simulink model "gofa_robot"  (R2023a)
settings: Solver=FixedStepAuto  StartTime=0.0  StopTime=11  FixedStep=0.001  RelTol=1e-3
undefined symbols (not defined in the file or in its folder): X, Y, Z
libraries: sm_lib x58, nesl_utility x10, slpidlib x3
(part 5 of 7)

== matlab function gofa_robot/gofa_FK_var ==
  data: x output; q1 input; y output; q2 input; q3 input; q4 input; q5 input; q6 input; z output; R output
function [x,y,z,R] = fcn(q1,q2,q3,q4,q5,q6)
d1 = 0.265;
d4 =0.47;
dee =0.101;
l3=0.444;
l4=0.110;
l6=0.08;
R=zeros(3,3);

R(1,1)= (24678615572571482867467662723121*cos(q6)*(cos(q5)*(cos(q3)*(cos(q1)*sin(q2 + pi/2) + (4967757600021511*cos(q2 + pi/2)*sin(q1))/81129638414606681695789005144064) - (4967757600021511*sin(q1))/81129638414606681695789005144064 + sin(q3)*(cos(q1)*cos(q2 + pi/2) - (4967757600021511*sin(q1)*sin(q2 + pi/2))/81129638414606681695789005144064)) + (4967757600021511*cos(q5)*(cos(q4)*sin(q1) + (4967757600021511*cos(q4)*(cos(q3)*(cos(q1)*sin(q2 + pi/2) + (4967757600021511*cos(q2 + pi/2)*sin(q1))/81129638414606681695789005144064) + sin(q3)*(cos(q1)*cos(q2 + pi/2) - (4967757600021511*sin(q1)*sin(q2 + pi/2))/81129638414606681695789005144064)))/81129638414606681695789005144064 + sin(q4)*(cos(q3)*(cos(q1)*cos(q2 + pi/2) - (4967757600021511*sin(q1)*sin(q2 + pi/2))/81129638414606681695789005144064) - sin(q3)*(cos(q1)*sin(q2 + pi/2) + (4967757600021511*cos(q2 + pi/2)*sin(q1))/81129638414606681695789005144064))))/81129638414606681695789005144064 - sin(q5)*(sin(q1)*sin(q4) - cos(q4)*(cos(q3)*(cos(q1)*cos(q2 + pi/2) - (4967757600021511*sin(q1)*sin(q2 + pi/2))/81129638414606681695789005144064) - sin(q3)*(cos(q1)*sin(q2 + pi/2) + (4967757600021511*cos(q2 + pi/2)*sin(q1))/81129638414606681695789005144064)) + (4967757600021511*sin(q4)*(cos(q3)*(cos(q1)*sin(q2 + pi/2) + (4967757600021511*cos(q2 + pi/2)*sin(q1))/81129638414606681695789005144064) + sin(q3)*(cos(q1)*cos(q2 + pi/2) - (4967757600021511*sin(q1)*sin(q2 + pi/2))/81129638414606681695789005144064)))/81129638414606681695789005144064)))/3291009114642412084309938365114701009965471731267159726697218048 - cos(q6)*(sin(q5)*(cos(q3)*(cos(q1)*sin(q2 + pi/2) + (4967757600021511*cos(q2 + pi/2)*sin(q1))/81129638414606681695789005144064) - (4967757600021511*sin(q1))/81129638414606681695789005144064 + sin(q3)*(cos(q1)*cos(q2 + pi/2) - (4967757600021511*sin(q1)*sin(q2 + pi/2))/81129638414606681695789005144064)) + (4967757600021511*sin(q5)*(cos(q4)*sin(q1) + (4967757600021511*cos(q4)*(cos(q3)*(cos(q1)*sin(q2 + pi/2) + (4967757600021511*cos(q2 + pi/2)*sin(q1))/81129638414606681695789005144064) + sin(q3)*(cos(q1)*cos(q2 + pi/2) - (4967757600021511*sin(q1)*sin(q2 + pi/2))/81129638414606681695789005144064)))/81129638414606681695789005144064 + sin(q4)*(cos(q3)*(cos(q1)*cos(q2 + pi/2) - (4967757600021511*sin(q1)*sin(q2 + pi/2))/81129638414606681695789005144064) - sin(q3)*(cos(q1)*sin(q2 + pi/2) + (4967757600021511*cos(q2 + pi/2)*sin(q1))/81129638414606681695789005144064))))/81129638414606681695789005144064 + cos(q5)*(sin(q1)*sin(q4) - cos(q4)*(cos(q3)*(cos(q1)*cos(q2 + pi/2) - (4967757600021511*sin(q1)*sin(q2 + pi/2))/81129638414606681695789005144064) - sin(q3)*(cos(q1)*sin(q2 + pi/2) + (4967757600021511*cos(q2 + pi/2)*sin(q1))/81129638414606681695789005144064)) + (4967757600021511*sin(q4)*(cos(q3)*(cos(q1)*sin(q2 + pi/2) + (4967757600021511*cos(q2 + pi/2)*sin(q1))/81129638414606681695789005144064) + sin(q3)*(cos(q1)*cos(q2 + pi/2) - (4967757600021511*sin(q1)*sin(q2 + pi/2))/81129638414606681695789005144064)))/81129638414606681695789005144064)) - (4967757600021511*sin(q6)*(cos(q5)*(cos(q3)*(cos(q1)*sin(q2 + pi/2) + (4967757600021511*cos(q2 + pi/2)*sin(q1))/81129638414606681695789005144064) - (4967757600021511*sin(q1))/81129638414606681695789005144064 + sin(q3)*(cos(q1)*cos(q2 + pi/2) - (4967757600021511*sin(q1)*sin(q2 + pi/2))/81129638414606681695789005144064)) + (4967757600021511*cos(q5)*(cos(q4)*sin(q1) + (4967757600021511*cos(q4)*(cos(q3)*(cos(q1)*sin(q2 + pi/2) + (4967757600021511*cos(q2 + pi/2)*sin(q1))/81129638414606681695789005144064) + sin(q3)*(cos(q1)*cos(q2 + pi/2) - (4967757600021511*sin(q1)*sin(q2 + pi/2))/81129638414606681695789005144064)))/81129638414606681695789005144064 + sin(q4)*(cos(q3)*(cos(q1)*cos(q2 + pi/2) - (4967757600021511*sin(q1)*sin(q2 + pi/2))/81129638414606681695789005144064) - sin(q3)*(cos(q1)*sin(q2 + pi/2) + (4967757600021511*cos(q2 + pi/2)*sin(q1))/81129638414606681695789005144064))))/81129638414606681695789005144064 - sin(q5)*(sin(q1)*sin(q4) - cos(q4)*(cos(q3)*(cos(q1)*cos(q2 + pi/2) - (4967757600021511*sin(q1)*sin(q2 + pi/2))/81129638414606681695789005144064) - sin(q3)*(cos(q1)*sin(q2 + pi/2) + (4967757600021511*cos(q2 + pi/2)*sin(q1))/81129638414606681695789005144064)) + (4967757600021511*sin(q4)*(cos(q3)*(cos(q1)*sin(q2 + pi/2) + (4967757600021511*cos(q2 + pi/2)*sin(q1))/81129638414606681695789005144064) + sin(q3)*(cos(q1)*cos(q2 + pi/2) - (4967757600021511*sin(q1)*sin(q2 + pi/2))/81129638414606681695789005144064)))/81129638414606681695789005144064)))/81129638414606681695789005144064 - (4967757600021511*sin(q6)*(sin(q5)*(cos(q3)*(cos(q1)*sin(q2 + pi/2) + (4967757600021511*cos(q2 + pi/2)*sin(q1))/81129638414606681695789005144064) - (4967757600021511*sin(q1))/81129638414606681695789005144064 + sin(q3)*(cos(q1)*cos(q2 + pi/2) - (4967757600021511*sin(q1)*sin(q2 + pi/2))/81129638414606681695789005144064)) + (4967757600021511*sin(q5)*(cos(q4)*sin(q1) + (4967757600021511*cos(q4)*(cos(q3)*(cos(q1)*sin(q2 + pi/2) + (4967757600021511*cos(q2 + pi/2)*sin(q1))/81129638414606681695789005144064) + sin(q3)*(cos(q1)*cos(q2 + pi/2) - (4967757600021511*sin(q1)*sin(q2 + pi/2))/81129638414606681695789005144064)))/81129638414606681695789005144064 + sin(q4)*(cos(q3)*(cos(q1)*cos(q2 + pi/2) - (4967757600021511*sin(q1)*sin(q2 + pi/2))/81129638414606681695789005144064) - sin(q3)*(cos(q1)*sin(q2 + pi/2) + (4967757600021511*cos(q2 + pi/2)*sin(q1))/81129638414606681695789005144064))))/81129638414606681695789005144064 + cos(q5)*(sin(q1)*sin(q4) - cos(q4)*(cos(q3)*(cos(q1)*cos(q2 + pi/2) - (4967757600021511*sin(q1)*sin(q2 + pi/2))/81129638414606681695789005144064) - sin(q3)*(cos(q1)*sin(q2 + pi/2) + (4967757600021511*cos(q2 + pi/2)*sin(q1))/81129638414606681695789005144064)) + (4967757600021511*sin(q4)*(cos(q3)*(cos(q1)*sin(q2 + pi/2) + (4967757600021511*cos(q2 + pi/2)*sin(q1))/81129638414606681695789005144064) + sin(q3)*(cos(q1)*cos(q2 + pi/2) - (4967757600021511*sin(q1)*sin(q2 + pi/2))/81129638414606681695789005144064)))/81129638414606681695789005144064)))/40564819207303340847894502572032 + (4967757600021511*cos(q6)*((24678615572571482867467662723121*sin(q1))/6582018229284824168619876730229402019930943462534319453394436096 - (4967757600021511*cos(q3)*(cos(q1)*sin(q2 + pi/2) + (4967757600021511*cos(q2 + pi/2)*sin(q1))/81129638414606681695789005144064))/81129638414606681695789005144064 + cos(q4)*sin(q1) - (4967757600021511*sin(q3)*(cos(q1)*cos(q2 + pi/2) - (4967757600021511*sin(q1)*sin(q2 + pi/2))/81129638414606681695789005144064))/81129638414606681695789005144064 + (4967757600021511*cos(q4)*(cos(q3)*(cos(q1)*sin(q2 + pi/2) + (4967757600021511*cos(q2 + pi/2)*sin(q1))/81129638414606681695789005144064) + sin(q3)*(cos(q1)*cos(q2 + pi/2) - (4967757600021511*sin(q1)*sin(q2 + pi/2))/81129638414606681695789005144064)))/81129638414606681695789005144064 + sin(q4)*(cos(q3)*(cos(q1)*cos(q2 + pi/2) - (4967757600021511*sin(q1)*sin(q2 + pi/2))/81129638414606681695789005144064) - sin(q3)*(cos(q1)*sin(q2 + pi/2) + (4967757600021511*cos(q2 + pi/2)*sin(q1))/81129638414606681695789005144064))))/40564819207303340847894502572032 - sin(q6)*((24678615572571482867467662723121*sin(q1))/6582018229284824168619876730229402019930943462534319453394436096 - (4967757600021511*cos(q3)*(cos(q1)*sin(q2 + pi/2) + (4967757600021511*cos(q2 + pi/2)*sin(q1))/81129638414606681695789005144064))/81129638414606681695789005144064 + cos(q4)*sin(q1) - (4967757600021511*sin(q3)*(cos(q1)*cos(q2 + pi/2) - (4967757600021511*sin(q1)*sin(q2 + pi/2))/81129638414606681695789005144064))/81129638414606681695789005144064 + (4967757600021511*cos(q4)*(cos(q3)*(cos(q1)*sin(q2 + pi/2) + (4967757600021511*cos(q2 + pi/2)*sin(q1))/81129638414606681695789005144064) + sin(q3)*(cos(q1)*cos(q2 + pi/2) - (4967757600021511*sin(q1)*sin(q2 + pi/2))/81129638414606681695789005144064)))/81129638414606681695789005144064 + sin(q4)*(cos(q3)*(cos(q1)*cos(q2 + pi/2) - (4967757600021511*sin(q1)*sin(q2 + pi/2))/81129638414606681695789005144064) - sin(q3)*(cos(q1)*sin(q2 + pi/2) + (4967757600021511*cos(q2 + pi/2)*sin(q1))/81129638414606681695789005144064)));
R(1,2)= sin(q6)*(sin(q5)*(cos(q3)*(cos(q1)*sin(q2 + pi/2) + (4967757600021511*cos(q2 + pi/2)*sin(q1))/81129638414606681695789005144064) - (4967757600021511*sin(q1))/81129638414606681695789005144064 + sin(q3)*(cos(q1)*cos(q2 + pi/2) - (4967757600021511*sin(q1)*sin(q2 + pi/2))/81129638414606681695789005144064)) + (4967757600021511*sin(q5)*(cos(q4)*sin(q1) + (4967757600021511*cos(q4)*(cos(q3)*(cos(q1)*sin(q2 + pi/2) + (4967757600021511*cos(q2 + pi/2)*sin(q1))/81129638414606681695789005144064) + sin(q3)*(cos(q1)*cos(q2 + pi/2) - (4967757600021511*sin(q1)*sin(q2 + pi/2))/81129638414606681695789005144064)))/81129638414606681695789005144064 + sin(q4)*(cos(q3)*(cos(q1)*cos(q2 + pi/2) - (4967757600021511*sin(q1)*sin(q2 + pi/2))/81129638414606681695789005144064) - sin(q3)*(cos(q1)*sin(q2 + pi/2) + (4967757600021511*cos(q2 + pi/2)*sin(q1))/81129638414606681695789005144064))))/81129638414606681695789005144064 + cos(q5)*(sin(q1)*sin(q4) - cos(q4)*(cos(q3)*(cos(q1)*cos(q2 + pi/2) - (4967757600021511*sin(q1)*sin(q2 + pi/2))/81129638414606681695789005144064) - sin(q3)*(cos(q1)*sin(q2 + pi/2) + (4967757600021511*cos(q2 + pi/2)*sin(q1))/81129638414606681695789005144064)) + (4967757600021511*sin(q4)*(cos(q3)*(cos(q1)*sin(q2 + pi/2) + (4967757600021511*cos(q2 + pi/2)*sin(q1))/81129638414606681695789005144064) + sin(q3)*(cos(q1)*cos(q2 + pi/2) - (4967757600021511*sin(q1)*sin(q2 + pi/2))/81129638414606681695789005144064)))/81129638414606681695789005144064)) - (4967757600021511*cos(q6)*(sin(q5)*(cos(q3)*(cos(q1)*sin(q2 + pi/2) + (4967757600021511*cos(q2 + pi/2)*sin(q1))/81129638414606681695789005144064) - (4967757600021511*sin(q1))/81129638414606681695789005144064 + sin(q3)*(cos(q1)*cos(q2 + pi/2) - (4967757600021511*sin(q1)*sin(q2 + pi/2))/81129638414606681695789005144064)) + (4967757600021511*sin(q5)*(cos(q4)*sin(q1) + (4967757600021511*cos(q4)*(cos(q3)*(cos(q1)*sin(q2 + pi/2) + (4967757600021511*cos(q2 + pi/2)*sin(q1))/81129638414606681695789005144064) + sin(q3)*(cos(q1)*cos(q2 + pi/2) - (4967757600021511*sin(q1)*sin(q2 + pi/2))/81129638414606681695789005144064)))/81129638414606681695789005144064 + sin(q4)*(cos(q3)*(cos(q1)*cos(q2 + pi/2) - (4967757600021511*sin(q1)*sin(q2 + pi/2))/81129638414606681695789005144064) - sin(q3)*(cos(q1)*sin(q2 + pi/2) + (4967757600021511*cos(q2 + pi/2)*sin(q1))/81129638414606681695789005144064))))/81129638414606681695789005144064 + cos(q5)*(sin(q1)*sin(q4) - cos(q4)*(cos(q3)*(cos(q1)*cos(q2 + pi/2) - (4967757600021511*sin(q1)*sin(q2 + pi/2))/81129638414606681695789005144064) - sin(q3)*(cos(q1)*sin(q2 + pi/2) + (4967757600021511*cos(q2 + pi/2)*sin(q1))/81129638414606681695789005144064)) + (4967757600021511*sin(q4)*(cos(q3)*(cos(q1)*sin(q2 + pi/2) + (4967757600021511*cos(q2 + pi/2)*sin(q1))/81129638414606681695789005144064) + sin(q3)*(cos(q1)*cos(q2 + pi/2) - (4967757600021511*sin(q1)*sin(q2 + pi/2))/81129638414606681695789005144064)))/81129638414606681695789005144064)))/40564819207303340847894502572032 - (24678615572571482867467662723121*sin(q6)*(cos(q5)*(cos(q3)*(cos(q1)*sin(q2 + pi/2) + (4967757600021511*cos(q2 + pi/2)*sin(q1))/81129638414606681695789005144064) - (4967757600021511*sin(q1))/81129638414606681695789005144064 + sin(q3)*(cos(q1)*cos(q2 + pi/2) - (4967757600021511*sin(q1)*sin(q2 + pi/2))/81129638414606681695789005144064)) + (4967757600021511*cos(q5)*(cos(q4)*sin(q1) + (4967757600021511*cos(q4)*(cos(q3)*(cos(q1)*sin(q2 + pi/2) + (4967757600021511*cos(q2 + pi/2)*sin(q1))/81129638414606681695789005144064) + sin(q3)*(cos(q1)*cos(q2 + pi/2) - (4967757600021511*sin(q1)*sin(q2 + pi/2))/81129638414606681695789005144064)))/81129638414606681695789005144064 + sin(q4)*(cos(q3)*(cos(q1)*cos(q2 + pi/2) - (4967757600021511*sin(q1)*sin(q2 + pi/2))/81129638414606681695789005144064) - sin(q3)*(cos(q1)*sin(q2 + pi/2) + (4967757600021511*cos(q2 + pi/2)*sin(q1))/81129638414606681695789005144064))))/81129638414606681695789005144064 - sin(q5)*(sin(q1)*sin(q4) - cos(q4)*(cos(q3)*(cos(q1)*cos(q2 + pi/2) - (4967757600021511*sin(q1)*sin(q2 + pi/2))/81129638414606681695789005144064) - sin(q3)*(cos(q1)*sin(q2 + pi/2) + (4967757600021511*cos(q2 + pi/2)*sin(q1))/81129638414606681695789005144064)) + (4967757600021511*sin(q4)*(cos(q3)*(cos(q1)*sin(q2 + pi/2) + (4967757600021511*cos(q2 + pi/2)*sin(q1))/81129638414606681695789005144064) + sin(q3)*(cos(q1)*cos(q2 + pi/2) - (4967757600021511*sin(q1)*sin(q2 + pi/2))/81129638414606681695789005144064)))/81129638414606681695789005144064)))/3291009114642412084309938365114701009965471731267159726697218048 - (4967757600021511*cos(q6)*(cos(q5)*(cos(q3)*(cos(q1)*sin(q2 + pi/2) + (4967757600021511*cos(q2 + pi/2)*sin(q1))/81129638414606681695789005144064) - (4967757600021511*sin(q1))/81129638414606681695789005144064 + sin(q3)*(cos(q1)*cos(q2 + pi/2) - (4967757600021511*sin(q1)*sin(q2 + pi/2))/81129638414606681695789005144064)) + (4967757600021511*cos(q5)*(cos(q4)*sin(q1) + (4967757600021511*cos(q4)*(cos(q3)*(cos(q1)*sin(q2 + pi/2) + (4967757600021511*cos(q2 + pi/2)*sin(q1))/81129638414606681695789005144064) + sin(q3)*(cos(q1)*cos(q2 + pi/2) - (4967757600021511*sin(q1)*sin(q2 + pi/2))/81129638414606681695789005144064)))/81129638414606681695789005144064 + sin(q4)*(cos(q3)*(cos(q1)*cos(q2 + pi/2) - (4967757600021511*sin(q1)*sin(q2 + pi/2))/81129638414606681695789005144064) - sin(q3)*(cos(q1)*sin(q2 + pi/2) + (4967757600021511*cos(q2 + pi/2)*sin(q1))/81129638414606681695789005144064))))/81129638414606681695789005144064 - sin(q5)*(sin(q1)*sin(q4) - cos(q4)*(cos(q3)*(cos(q1)*cos(q2 + pi/2) - (4967757600021511*sin(q1)*sin(q2 + pi/2))/81129638414606681695789005144064) - sin(q3)*(cos(q1)*sin(q2 + pi/2) + (4967757600021511*cos(q2 + pi/2)*sin(q1))/81129638414606681695789005144064)) + (4967757600021511*sin(q4)*(cos(q3)*(cos(q1)*sin(q2 + pi/2) + (4967757600021511*cos(q2 + pi/2)*sin(q1))/81129638414606681695789005144064) + sin(q3)*(cos(q1)*cos(q2 + pi/2) - (4967757600021511*sin(q1)*sin(q2 + pi/2))/81129638414606681695789005144064)))/81129638414606681695789005144064)))/81129638414606681695789005144064 - cos(q6)*((24678615572571482867467662723121*sin(q1))/6582018229284824168619876730229402019930943462534319453394436096 - (4967757600021511*cos(q3)*(cos(q1)*sin(q2 + pi/2) + (4967757600021511*cos(q2 + pi/2)*sin(q1))/81129638414606681695789005144064))/81129638414606681695789005144064 + cos(q4)*sin(q1) - (4967757600021511*sin(q3)*(cos(q1)*cos(q2 + pi/2) - (4967757600021511*sin(q1)*sin(q2 + pi/2))/81129638414606681695789005144064))/81129638414606681695789005144064 + (4967757600021511*cos(q4)*(cos(q3)*(cos(q1)*sin(q2 + pi/2) + (4967757600021511*cos(q2 + pi/2)*sin(q1))/81129638414606681695789005144064) + sin(q3)*(cos(q1)*cos(q2 + pi/2) - (4967757600021511*sin(q1)*sin(q2 + pi/2))/81129638414606681695789005144064)))/81129638414606681695789005144064 + sin(q4)*(cos(q3)*(cos(q1)*cos(q2 + pi/2) - (4967757600021511*sin(q1)*sin(q2 + pi/2))/81129638414606681695789005144064) - sin(q3)*(cos(q1)*sin(q2 + pi/2) + (4967757600021511*cos(q2 + pi/2)*sin(q1))/81129638414606681695789005144064))) - (4967757600021511*sin(q6)*((24678615572571482867467662723121*sin(q1))/6582018229284824168619876730229402019930943462534319453394436096 - (4967757600021511*cos(q3)*(cos(q1)*sin(q2 + pi/2) + (4967757600021511*cos(q2 + pi/2)*sin(q1))/81129638414606681695789005144064))/81129638414606681695789005144064 + cos(q4)*sin(q1) - (4967757600021511*sin(q3)*(cos(q1)*cos(q2 + pi/2) - (4967757600021511*sin(q1)*sin(q2 + pi/2))/81129638414606681695789005144064))/81129638414606681695789005144064 + (4967757600021511*cos(q4)*(cos(q3)*(cos(q1)*sin(q2 + pi/2) + (4967757600021511*cos(q2 + pi/2)*sin(q1))/81129638414606681695789005144064) + sin(q3)*(cos(q1)*cos(q2 + pi/2) - (4967757600021511*sin(q1)*sin(q2 + pi/2))/81129638414606681695789005144064)))/81129638414606681695789005144064 + sin(q4)*(cos(q3)*(cos(q1)*cos(q2 + pi/2) - (4967757600021511*sin(q1)*sin(q2 + pi/2))/81129638414606681695789005144064) - sin(q3)*(cos(q1)*sin(q2 + pi/2) + (4967757600021511*cos(q2 + pi/2)*sin(q1))/81129638414606681695789005144064))))/40564819207303340847894502572032;
R(1,3)= sin(q6)*(sin(q5)*(cos(q3)*(cos(q1)*sin(q2 + pi/2) + (4967757600021511*cos(q2 + pi/2)*sin(q1))/81129638414606681695789005144064) - (4967757600021511*sin(q1))/81129638414606681695789005144064 + sin(q3)*(cos(q1)*cos(q2 + pi/2) - (4967757600021511*sin(q1)*sin(q2 + pi/2))/81129638414606681695789005144064)) + (4967757600021511*sin(q5)*(cos(q4)*sin(q1) + (4967757600021511*cos(q4)*(cos(q3)*(cos(q1)*sin(q2 + pi/2) + (4967757600021511*cos(q2 + pi/2)*sin(q1))/81129638414606681695789005144064) + sin(q3)*(cos(q1)*cos(q2 + pi/2) - (4967757600021511*sin(q1)*sin(q2 + pi/2))/81129638414606681695789005144064)))/81129638414606681695789005144064 + sin(q4)*(cos(q3)*(cos(q1)*cos(q2 + pi/2) - (4967757600021511*sin(q1)*sin(q2 + pi/2))/81129638414606681695789005144064) - sin(q3)*(cos(q1)*sin(q2 + pi/2) + (4967757600021511*cos(q2 + pi/2)*sin(q1))/81129638414606681695789005144064))))/81129638414606681695789005144064 + cos(q5)*(sin(q1)*sin(q4) - cos(q4)*(cos(q3)*(cos(q1)*cos(q2 + pi/2) - (4967757600021511*sin(q1)*sin(q2 + pi/2))/81129638414606681695789005144064) - sin(q3)*(cos(q1)*sin(q2 + pi/2) + (4967757600021511*cos(q2 + pi/2)*sin(q1))/81129638414606681695789005144064)) + (4967757600021511*sin(q4)*(cos(q3)*(cos(q1)*sin(q2 + pi/2) + (4967757600021511*cos(q2 + pi/2)*sin(q1))/81129638414606681695789005144064) + sin(q3)*(cos(q1)*cos(q2 + pi/2) - (4967757600021511*sin(q1)*sin(q2 + pi/2))/81129638414606681695789005144064)))/81129638414606681695789005144064)) - (4967757600021511*cos(q6)*(sin(q5)*(cos(q3)*(cos(q1)*sin(q2 + pi/2) + (4967757600021511*cos(q2 + pi/2)*sin(q1))/81129638414606681695789005144064) - (4967757600021511*sin(q1))/81129638414606681695789005144064 + sin(q3)*(cos(q1)*cos(q2 + pi/2) - (4967757600021511*sin(q1)*sin(q2 + pi/2))/81129638414606681695789005144064)) + (4967757600021511*sin(q5)*(cos(q4)*sin(q1) + (4967757600021511*cos(q4)*(cos(q3)*(cos(q1)*sin(q2 + pi/2) + (4967757600021511*cos(q2 + pi/2)*sin(q1))/81129638414606681695789005144064) + sin(q3)*(cos(q1)*cos(q2 + pi/2) - (4967757600021511*sin(q1)*sin(q2 + pi/2))/81129638414606681695789005144064)))/81129638414606681695789005144064 + sin(q4)*(cos(q3)*(cos(q1)*cos(q2 + pi/2) - (4967757600021511*sin(q1)*sin(q2 + pi/2))/81129638414606681695789005144064) - sin(q3)*(cos(q1)*sin(q2 + pi/2) + (4967757600021511*cos(q2 + pi/2)*sin(q1))/81129638414606681695789005144064))))/81129638414606681695789005144064 + cos(q5)*(sin(q1)*sin(q4) - cos(q4)*(cos(q3)*(cos(q1)*cos(q2 + pi/2) - (4967757600021511*sin(q1)*sin(q2 + pi/2))/81129638414606681695789005144064) - sin(q3)*(cos(q1)*sin(q2 + pi/2) + (4967757600021511*cos(q2 + pi/2)*sin(q1))/81129638414606681695789005144064)) + (4967757600021511*sin(q4)*(cos(q3)*(cos(q1)*sin(q2 + pi/2) + (4967757600021511*cos(q2 + pi/2)*sin(q1))/81129638414606681695789005144064) + sin(q3)*(cos(q1)*cos(q2 + pi/2) - (4967757600021511*sin(q1)*sin(q2 + pi/2))/81129638414606681695789005144064)))/81129638414606681695789005144064)))/40564819207303340847894502572032 - (24678615572571482867467662723121*sin(q6)*(cos(q5)*(cos(q3)*(cos(q1)*sin(q2 + pi/2) + (4967757600021511*cos(q2 + pi/2)*sin(q1))/81129638414606681695789005144064) - (4967757600021511*sin(q1))/81129638414606681695789005144064 + sin(q3)*(cos(q1)*cos(q2 + pi/2) - (4967757600021511*sin(q1)*sin(q2 + pi/2))/81129638414606681695789005144064)) + (4967757600021511*cos(q5)*(cos(q4)*sin(q1) + (4967757600021511*cos(q4)*(cos(q3)*(cos(q1)*sin(q2 + pi/2) + (4967757600021511*cos(q2 + pi/2)*sin(q1))/81129638414606681695789005144064) + sin(q3)*(cos(q1)*cos(q2 + pi/2) - (4967757600021511*sin(q1)*sin(q2 + pi/2))/81129638414606681695789005144064)))/81129638414606681695789005144064 + sin(q4)*(cos(q3)*(cos(q1)*cos(q2 + pi/2) - (4967757600021511*sin(q1)*sin(q2 + pi/2))/81129638414606681695789005144064) - sin(q3)*(cos(q1)*sin(q2 + pi/2) + (4967757600021511*cos(q2 + pi/2)*sin(q1))/81129638414606681695789005144064))))/81129638414606681695789005144064 - sin(q5)*(sin(q1)*sin(q4) - cos(q4)*(cos(q3)*(cos(q1)*cos(q2 + pi/2) - (4967757600021511*sin(q1)*sin(q2 + pi/2))/81129638414606681695789005144064) - sin(q3)*(cos(q1)*sin(q2 + pi/2) + (4967757600021511*cos(q2 + pi/2)*sin(q1))/81129638414606681695789005144064)) + (4967757600021511*sin(q4)*(cos(q3)*(cos(q1)*sin(q2 + pi/2) + (4967757600021511*cos(q2 + pi/2)*sin(q1))/81129638414606681695789005144064) + sin(q3)*(cos(q1)*cos(q2 + pi/2) - (4967757600021511*sin(q1)*sin(q2 + pi/2))/81129638414606681695789005144064)))/81129638414606681695789005144064)))/3291009114642412084309938365114701009965471731267159726697218048 - (4967757600021511*cos(q6)*(cos(q5)*(cos(q3)*(cos(q1)*sin(q2 + pi/2) + (4967757600021511*cos(q2 + pi/2)*sin(q1))/81129638414606681695789005144064) - (4967757600021511*sin(q1))/81129638414606681695789005144064 + sin(q3)*(cos(q1)*cos(q2 + pi/2) - (4967757600021511*sin(q1)*sin(q2 + pi/2))/81129638414606681695789005144064)) + (4967757600021511*cos(q5)*(cos(q4)*sin(q1) + (4967757600021511*cos(q4)*(cos(q3)*(cos(q1)*sin(q2 + pi/2) + (4967757600021511*cos(q2 + pi/2)*sin(q1))/81129638414606681695789005144064) + sin(q3)*(cos(q1)*cos(q2 + pi/2) - (4967757600021511*sin(q1)*sin(q2 + pi/2))/81129638414606681695789005144064)))/81129638414606681695789005144064 + sin(q4)*(cos(q3)*(cos(q1)*cos(q2 + pi/2) - (4967757600021511*sin(q1)*sin(q2 + pi/2))/81129638414606681695789005144064) - sin(q3)*(cos(q1)*sin(q2 + pi/2) + (4967757600021511*cos(q2 + pi/2)*sin(q1))/81129638414606681695789005144064))))/81129638414606681695789005144064 - sin(q5)*(sin(q1)*sin(q4) - cos(q4)*(cos(q3)*(cos(q1)*cos(q2 + pi/2) - (4967757600021511*sin(q1)*sin(q2 + pi/2))/81129638414606681695789005144064) - sin(q3)*(cos(q1)*sin(q2 + pi/2) + (4967757600021511*cos(q2 + pi/2)*sin(q1))/81129638414606681695789005144064)) + (4967757600021511*sin(q4)*(cos(q3)*(cos(q1)*sin(q2 + pi/2) + (4967757600021511*cos(q2 + pi/2)*sin(q1))/81129638414606681695789005144064) + sin(q3)*(cos(q1)*cos(q2 + pi/2) - (4967757600021511*sin(q1)*sin(q2 + pi/2))/81129638414606681695789005144064)))/81129638414606681695789005144064)))/81129638414606681695789005144064 - cos(q6)*((24678615572571482867467662723121*sin(q1))/6582018229284824168619876730229402019930943462534319453394436096 - (4967757600021511*cos(q3)*(cos(q1)*sin(q2 + pi/2) + (4967757600021511*cos(q2 + pi/2)*sin(q1))/81129638414606681695789005144064))/81129638414606681695789005144064 + cos(q4)*sin(q1) - (4967757600021511*sin(q3)*(cos(q1)*cos(q2 + pi/2) - (4967757600021511*sin(q1)*sin(q2 + pi/2))/81129638414606681695789005144064))/81129638414606681695789005144064 + (4967757600021511*cos(q4)*(cos(q3)*(cos(q1)*sin(q2 + pi/2) + (4967757600021511*cos(q2 + pi/2)*sin(q1))/81129638414606681695789005144064) + sin(q3)*(cos(q1)*cos(q2 + pi/2) - (4967757600021511*sin(q1)*sin(q2 + pi/2))/81129638414606681695789005144064)))/81129638414606681695789005144064 + sin(q4)*(cos(q3)*(cos(q1)*cos(q2 + pi/2) - (4967757600021511*sin(q1)*sin(q2 + pi/2))/81129638414606681695789005144064) - sin(q3)*(cos(q1)*sin(q2 + pi/2) + (4967757600021511*cos(q2 + pi/2)*sin(q1))/81129638414606681695789005144064))) - (4967757600021511*sin(q6)*((24678615572571482867467662723121*sin(q1))/6582018229284824168619876730229402019930943462534319453394436096 - (4967757600021511*cos(q3)*(cos(q1)*sin(q2 + pi/2) + (4967757600021511*cos(q2 + pi/2)*sin(q1))/81129638414606681695789005144064))/81129638414606681695789005144064 + cos(q4)*sin(q1) - (4967757600021511*sin(q3)*(cos(q1)*cos(q2 + pi/2) - (4967757600021511*sin(q1)*sin(q2 + pi/2))/81129638414606681695789005144064))/81129638414606681695789005144064 + (4967757600021511*cos(q4)*(cos(q3)*(cos(q1)*sin(q2 + pi/2) + (4967757600021511*cos(q2 + pi/2)*sin(q1))/81129638414606681695789005144064) + sin(q3)*(cos(q1)*cos(q2 + pi/2) - (4967757600021511*sin(q1)*sin(q2 + pi/2))/81129638414606681695789005144064)))/81129638414606681695789005144064 + sin(q4)*(cos(q3)*(cos(q1)*cos(q2 + pi/2) - (4967757600021511*sin(q1)*sin(q2 + pi/2))/81129638414606681695789005144064) - sin(q3)*(cos(q1)*sin(q2 + pi/2) + (4967757600021511*cos(q2 + pi/2)*sin(q1))/81129638414606681695789005144064))))/40564819207303340847894502572032;
R(2,1)= (24678615572571482867467662723121*cos(q6)*(cos(q5)*((4967757600021511*cos(q1))/81129638414606681695789005144064 - cos(q3)*((4967757600021511*cos(q1)*cos(q2 + pi/2))/81129638414606681695789005144064 - sin(q1)*sin(q2 + pi/2)) + sin(q3)*((4967757600021511*cos(q1)*sin(q2 + pi/2))/81129638414606681695789005144064 + cos(q2 + pi/2)*sin(q1))) - (4967757600021511*cos(q5)*(cos(q1)*cos(q4) + (4967757600021511*cos(q4)*(cos(q3)*((4967757600021511*cos(q1)*cos(q2 + pi/2))/81129638414606681695789005144064 - sin(q1)*sin(q2 + pi/2)) - sin(q3)*((4967757600021511*cos(q1)*sin(q2 + pi/2))/81129638414606681695789005144064 + cos(q2 + pi/2)*sin(q1))))/81129638414606681695789005144064 - sin(q4)*(cos(q3)*((4967757600021511*cos(q1)*sin(q2 + pi/2))/81129638414606681695789005144064 + cos(q2 + pi/2)*sin(q1)) + sin(q3)*((4967757600021511*cos(q1)*cos(q2 + pi/2))/81129638414606681695789005144064 - sin(q1)*sin(q2 + pi/2)))))/81129638414606681695789005144064 + sin(q5)*(cos(q1)*sin(q4) + cos(q4)*(cos(q3)*((4967757600021511*cos(q1)*sin(q2 + pi/2))/81129638414606681695789005144064 + cos(q2 + pi/2)*sin(q1)) + sin(q3)*((4967757600021511*cos(q1)*cos(q2 + pi/2))/81129638414606681695789005144064 - sin(q1)*sin(q2 + pi/2))) + (4967757600021511*sin(q4)*(cos(q3)*((4967757600021511*cos(q1)*cos(q2 + pi/2))/81129638414606681695789005144064 - sin(q1)*sin(q2 + pi/2)) - sin(q3)*((4967757600021511*cos(q1)*sin(q2 + pi/2))/81129638414606681695789005144064 + cos(q2 + pi/2)*sin(q1))))/81129638414606681695789005144064)))/3291009114642412084309938365114701009965471731267159726697218048 - (4967757600021511*sin(q6)*(cos(q5)*((4967757600021511*cos(q1))/81129638414606681695789005144064 - cos(q3)*((4967757600021511*cos(q1)*cos(q2 + pi/2))/81129638414606681695789005144064 - sin(q1)*sin(q2 + pi/2)) + sin(q3)*((4967757600021511*cos(q1)*sin(q2 + pi/2))/81129638414606681695789005144064 + cos(q2 + pi/2)*sin(q1))) - (4967757600021511*cos(q5)*(cos(q1)*cos(q4) + (4967757600021511*cos(q4)*(cos(q3)*((4967757600021511*cos(q1)*cos(q2 + pi/2))/81129638414606681695789005144064 - sin(q1)*sin(q2 + pi/2)) - sin(q3)*((4967757600021511*cos(q1)*sin(q2 + pi/2))/81129638414606681695789005144064 + cos(q2 + pi/2)*sin(q1))))/81129638414606681695789005144064 - sin(q4)*(cos(q3)*((4967757600021511*cos(q1)*sin(q2 + pi/2))/81129638414606681695789005144064 + cos(q2 + pi/2)*sin(q1)) + sin(q3)*((4967757600021511*cos(q1)*cos(q2 + pi/2))/81129638414606681695789005144064 - sin(q1)*sin(q2 + pi/2)))))/81129638414606681695789005144064 + sin(q5)*(cos(q1)*sin(q4) + cos(q4)*(cos(q3)*((4967757600021511*cos(q1)*sin(q2 + pi/2))/81129638414606681695789005144064 + cos(q2 + pi/2)*sin(q1)) + sin(q3)*((4967757600021511*cos(q1)*cos(q2 + pi/2))/81129638414606681695789005144064 - sin(q1)*sin(q2 + pi/2))) + (4967757600021511*sin(q4)*(cos(q3)*((4967757600021511*cos(q1)*cos(q2 + pi/2))/81129638414606681695789005144064 - sin(q1)*sin(q2 + pi/2)) - sin(q3)*((4967757600021511*cos(q1)*sin(q2 + pi/2))/81129638414606681695789005144064 + cos(q2 + pi/2)*sin(q1))))/81129638414606681695789005144064)))/81129638414606681695789005144064 + cos(q6)*(cos(q5)*(cos(q1)*sin(q4) + cos(q4)*(cos(q3)*((4967757600021511*cos(q1)*sin(q2 + pi/2))/81129638414606681695789005144064 + cos(q2 + pi/2)*sin(q1)) + sin(q3)*((4967757600021511*cos(q1)*cos(q2 + pi/2))/81129638414606681695789005144064 - sin(q1)*sin(q2 + pi/2))) + (4967757600021511*sin(q4)*(cos(q3)*((4967757600021511*cos(q1)*cos(q2 + pi/2))/81129638414606681695789005144064 - sin(q1)*sin(q2 + pi/2)) - sin(q3)*((4967757600021511*cos(q1)*sin(q2 + pi/2))/81129638414606681695789005144064 + cos(q2 + pi/2)*sin(q1))))/81129638414606681695789005144064) - sin(q5)*((4967757600021511*cos(q1))/81129638414606681695789005144064 - cos(q3)*((4967757600021511*cos(q1)*cos(q2 + pi/2))/81129638414606681695789005144064 - sin(q1)*sin(q2 + pi/2)) + sin(q3)*((4967757600021511*cos(q1)*sin(q2 + pi/2))/81129638414606681695789005144064 + cos(q2 + pi/2)*sin(q1))) + (4967757600021511*sin(q5)*(cos(q1)*cos(q4) + (4967757600021511*cos(q4)*(cos(q3)*((4967757600021511*cos(q1)*cos(q2 + pi/2))/81129638414606681695789005144064 - sin(q1)*sin(q2 + pi/2)) - sin(q3)*((4967757600021511*cos(q1)*sin(q2 + pi/2))/81129638414606681695789005144064 + cos(q2 + pi/2)*sin(q1))))/81129638414606681695789005144064 - sin(q4)*(cos(q3)*((4967757600021511*cos(q1)*sin(q2 + pi/2))/81129638414606681695789005144064 + cos(q2 + pi/2)*sin(q1)) + sin(q3)*((4967757600021511*cos(q1)*cos(q2 + pi/2))/81129638414606681695789005144064 - sin(q1)*sin(q2 + pi/2)))))/81129638414606681695789005144064) + (4967757600021511*sin(q6)*(cos(q5)*(cos(q1)*sin(q4) + cos(q4)*(cos(q3)*((4967757600021511*cos(q1)*sin(q2 + pi/2))/81129638414606681695789005144064 + cos(q2 + pi/2)*sin(q1)) + sin(q3)*((4967757600021511*cos(q1)*cos(q2 + pi/2))/81129638414606681695789005144064 - sin(q1)*sin(q2 + pi/2))) + (4967757600021511*sin(q4)*(cos(q3)*((4967757600021511*cos(q1)*cos(q2 + pi/2))/81129638414606681695789005144064 - sin(q1)*sin(q2 + pi/2)) - sin(q3)*((4967757600021511*cos(q1)*sin(q2 + pi/2))/81129638414606681695789005144064 + cos(q2 + pi/2)*sin(q1))))/81129638414606681695789005144064) - sin(q5)*((4967757600021511*cos(q1))/81129638414606681695789005144064 - cos(q3)*((4967757600021511*cos(q1)*cos(q2 + pi/2))/81129638414606681695789005144064 - sin(q1)*sin(q2 + pi/2)) + sin(q3)*((4967757600021511*cos(q1)*sin(q2 + pi/2))/81129638414606681695789005144064 + cos(q2 + pi/2)*sin(q1))) + (4967757600021511*sin(q5)*(cos(q1)*cos(q4) + (4967757600021511*cos(q4)*(cos(q3)*((4967757600021511*cos(q1)*cos(q2 + pi/2))/81129638414606681695789005144064 - sin(q1)*sin(q2 + pi/2)) - sin(q3)*((4967757600021511*cos(q1)*sin(q2 + pi/2))/81129638414606681695789005144064 + cos(q2 + pi/2)*sin(q1))))/81129638414606681695789005144064 - sin(q4)*(cos(q3)*((4967757600021511*cos(q1)*sin(q2 + pi/2))/81129638414606681695789005144064 + cos(q2 + pi/2)*sin(q1)) + sin(q3)*((4967757600021511*cos(q1)*cos(q2 + pi/2))/81129638414606681695789005144064 - sin(q1)*sin(q2 + pi/2)))))/81129638414606681695789005144064))/40564819207303340847894502572032 - (4967757600021511*cos(q6)*((24678615572571482867467662723121*cos(q1))/6582018229284824168619876730229402019930943462534319453394436096 + cos(q1)*cos(q4) - (4967757600021511*cos(q3)*((4967757600021511*cos(q1)*cos(q2 + pi/2))/81129638414606681695789005144064 - sin(q1)*sin(q2 + pi/2)))/81129638414606681695789005144064 + (4967757600021511*sin(q3)*((4967757600021511*cos(q1)*sin(q2 + pi/2))/81129638414606681695789005144064 + cos(q2 + pi/2)*sin(q1)))/81129638414606681695789005144064 + (4967757600021511*cos(q4)*(cos(q3)*((4967757600021511*cos(q1)*cos(q2 + pi/2))/81129638414606681695789005144064 - sin(q1)*sin(q2 + pi/2)) - sin(q3)*((4967757600021511*cos(q1)*sin(q2 + pi/2))/81129638414606681695789005144064 + cos(q2 + pi/2)*sin(q1))))/81129638414606681695789005144064 - sin(q4)*(cos(q3)*((4967757600021511*cos(q1)*sin(q2 + pi/2))/81129638414606681695789005144064 + cos(q2 + pi/2)*sin(q1)) + sin(q3)*((4967757600021511*cos(q1)*cos(q2 + pi/2))/81129638414606681695789005144064 - sin(q1)*sin(q2 + pi/2)))))/40564819207303340847894502572032 + sin(q6)*((24678615572571482867467662723121*cos(q1))/6582018229284824168619876730229402019930943462534319453394436096 + cos(q1)*cos(q4) - (4967757600021511*cos(q3)*((4967757600021511*cos(q1)*cos(q2 + pi/2))/81129638414606681695789005144064 - sin(q1)*sin(q2 + pi/2)))/81129638414606681695789005144064 + (4967757600021511*sin(q3)*((4967757600021511*cos(q1)*sin(q2 + pi/2))/81129638414606681695789005144064 + cos(q2 + pi/2)*sin(q1)))/81129638414606681695789005144064 + (4967757600021511*cos(q4)*(cos(q3)*((4967757600021511*cos(q1)*cos(q2 + pi/2))/81129638414606681695789005144064 - sin(q1)*sin(q2 + pi/2)) - sin(q3)*((4967757600021511*cos(q1)*sin(q2 + pi/2))/81129638414606681695789005144064 + cos(q2 + pi/2)*sin(q1))))/81129638414606681695789005144064 - sin(q4)*(cos(q3)*((4967757600021511*cos(q1)*sin(q2 + pi/2))/81129638414606681695789005144064 + cos(q2 + pi/2)*sin(q1)) + sin(q3)*((4967757600021511*cos(q1)*cos(q2 + pi/2))/81129638414606681695789005144064 - sin(q1)*sin(q2 + pi/2)))); 
R(2,2)= (4967757600021511*cos(q6)*(cos(q5)*(cos(q1)*sin(q4) + cos(q4)*(cos(q3)*((4967757600021511*cos(q1)*sin(q2 + pi/2))/81129638414606681695789005144064 + cos(q2 + pi/2)*sin(q1)) + sin(q3)*((4967757600021511*cos(q1)*cos(q2 + pi/2))/81129638414606681695789005144064 - sin(q1)*sin(q2 + pi/2))) + (4967757600021511*sin(q4)*(cos(q3)*((4967757600021511*cos(q1)*cos(q2 + pi/2))/81129638414606681695789005144064 - sin(q1)*sin(q2 + pi/2)) - sin(q3)*((4967757600021511*cos(q1)*sin(q2 + pi/2))/81129638414606681695789005144064 + cos(q2 + pi/2)*sin(q1))))/81129638414606681695789005144064) - sin(q5)*((4967757600021511*cos(q1))/81129638414606681695789005144064 - cos(q3)*((4967757600021511*cos(q1)*cos(q2 + pi/2))/81129638414606681695789005144064 - sin(q1)*sin(q2 + pi/2)) + sin(q3)*((4967757600021511*cos(q1)*sin(q2 + pi/2))/81129638414606681695789005144064 + cos(q2 + pi/2)*sin(q1))) + (4967757600021511*sin(q5)*(cos(q1)*cos(q4) + (4967757600021511*cos(q4)*(cos(q3)*((4967757600021511*cos(q1)*cos(q2 + pi/2))/81129638414606681695789005144064 - sin(q1)*sin(q2 + pi/2)) - sin(q3)*((4967757600021511*cos(q1)*sin(q2 + pi/2))/81129638414606681695789005144064 + cos(q2 + pi/2)*sin(q1))))/81129638414606681695789005144064 - sin(q4)*(cos(q3)*((4967757600021511*cos(q1)*sin(q2 + pi/2))/81129638414606681695789005144064 + cos(q2 + pi/2)*sin(q1)) + sin(q3)*((4967757600021511*cos(q1)*cos(q2 + pi/2))/81129638414606681695789005144064 - sin(q1)*sin(q2 + pi/2)))))/81129638414606681695789005144064))/40564819207303340847894502572032 - (24678615572571482867467662723121*sin(q6)*(cos(q5)*((4967757600021511*cos(q1))/81129638414606681695789005144064 - cos(q3)*((4967757600021511*cos(q1)*cos(q2 + pi/2))/81129638414606681695789005144064 - sin(q1)*sin(q2 + pi/2)) + sin(q3)*((4967757600021511*cos(q1)*sin(q2 + pi/2))/81129638414606681695789005144064 + cos(q2 + pi/2)*sin(q1))) - (4967757600021511*cos(q5)*(cos(q1)*cos(q4) + (4967757600021511*cos(q4)*(cos(q3)*((4967757600021511*cos(q1)*cos(q2 + pi/2))/81129638414606681695789005144064 - sin(q1)*sin(q2 + pi/2)) - sin(q3)*((4967757600021511*cos(q1)*sin(q2 + pi/2))/81129638414606681695789005144064 + cos(q2 + pi/2)*sin(q1))))/81129638414606681695789005144064 - sin(q4)*(cos(q3)*((4967757600021511*cos(q1)*sin(q2 + pi/2))/81129638414606681695789005144064 + cos(q2 + pi/2)*sin(q1)) + sin(q3)*((4967757600021511*cos(q1)*cos(q2 + pi/2))/81129638414606681695789005144064 - sin(q1)*sin(q2 + pi/2)))))/81129638414606681695789005144064 + sin(q5)*(cos(q1)*sin(q4) + cos(q4)*(cos(q3)*((4967757600021511*cos(q1)*sin(q2 + pi/2))/81129638414606681695789005144064 + cos(q2 + pi/2)*sin(q1)) + sin(q3)*((4967757600021511*cos(q1)*cos(q2 + pi/2))/81129638414606681695789005144064 - sin(q1)*sin(q2 + pi/2))) + (4967757600021511*sin(q4)*(cos(q3)*((4967757600021511*cos(q1)*cos(q2 + pi/2))/81129638414606681695789005144064 - sin(q1)*sin(q2 + pi/2)) - sin(q3)*((4967757600021511*cos(q1)*sin(q2 + pi/2))/81129638414606681695789005144064 + cos(q2 + pi/2)*sin(q1))))/81129638414606681695789005144064)))/3291009114642412084309938365114701009965471731267159726697218048 - (4967757600021511*cos(q6)*(cos(q5)*((4967757600021511*cos(q1))/81129638414606681695789005144064 - cos(q3)*((4967757600021511*cos(q1)*cos(q2 + pi/2))/81129638414606681695789005144064 - sin(q1)*sin(q2 + pi/2)) + sin(q3)*((4967757600021511*cos(q1)*sin(q2 + pi/2))/81129638414606681695789005144064 + cos(q2 + pi/2)*sin(q1))) - (4967757600021511*cos(q5)*(cos(q1)*cos(q4) + (4967757600021511*cos(q4)*(cos(q3)*((4967757600021511*cos(q1)*cos(q2 + pi/2))/81129638414606681695789005144064 - sin(q1)*sin(q2 + pi/2)) - sin(q3)*((4967757600021511*cos(q1)*sin(q2 + pi/2))/81129638414606681695789005144064 + cos(q2 + pi/2)*sin(q1))))/81129638414606681695789005144064 - sin(q4)*(cos(q3)*((4967757600021511*cos(q1)*sin(q2 + pi/2))/81129638414606681695789005144064 + cos(q2 + pi/2)*sin(q1)) + sin(q3)*((4967757600021511*cos(q1)*cos(q2 + pi/2))/81129638414606681695789005144064 - sin(q1)*sin(q2 + pi/2)))))/81129638414606681695789005144064 + sin(q5)*(cos(q1)*sin(q4) + cos(q4)*(cos(q3)*((4967757600021511*cos(q1)*sin(q2 + pi/2))/81129638414606681695789005144064 + cos(q2 + pi/2)*sin(q1)) + sin(q3)*((4967757600021511*cos(q1)*cos(q2 + pi/2))/81129638414606681695789005144064 - sin(q1)*sin(q2 + pi/2))) + (4967757600021511*sin(q4)*(cos(q3)*((4967757600021511*cos(q1)*cos(q2 + pi/2))/81129638414606681695789005144064 - sin(q1)*sin(q2 + pi/2)) - sin(q3)*((4967757600021511*cos(q1)*sin(q2 + pi/2))/81129638414606681695789005144064 + cos(q2 + pi/2)*sin(q1))))/81129638414606681695789005144064)))/81129638414606681695789005144064 - sin(q6)*(cos(q5)*(cos(q1)*sin(q4) + cos(q4)*(cos(q3)*((4967757600021511*cos(q1)*sin(q2 + pi/2))/81129638414606681695789005144064 + cos(q2 + pi/2)*sin(q1)) + sin(q3)*((4967757600021511*cos(q1)*cos(q2 + pi/2))/81129638414606681695789005144064 - sin(q1)*sin(q2 + pi/2))) + (4967757600021511*sin(q4)*(cos(q3)*((4967757600021511*cos(q1)*cos(q2 + pi/2))/81129638414606681695789005144064 - sin(q1)*sin(q2 + pi/2)) - sin(q3)*((4967757600021511*cos(q1)*sin(q2 + pi/2))/81129638414606681695789005144064 + cos(q2 + pi/2)*sin(q1))))/81129638414606681695789005144064) - sin(q5)*((4967757600021511*cos(q1))/81129638414606681695789005144064 - cos(q3)*((4967757600021511*cos(q1)*cos(q2 + pi/2))/81129638414606681695789005144064 - sin(q1)*sin(q2 + pi/2)) + sin(q3)*((4967757600021511*cos(q1)*sin(q2 + pi/2))/81129638414606681695789005144064 + cos(q2 + pi/2)*sin(q1))) + (4967757600021511*sin(q5)*(cos(q1)*cos(q4) + (4967757600021511*cos(q4)*(cos(q3)*((4967757600021511*cos(q1)*cos(q2 + pi/2))/81129638414606681695789005144064 - sin(q1)*sin(q2 + pi/2)) - sin(q3)*((4967757600021511*cos(q1)*sin(q2 + pi/2))/81129638414606681695789005144064 + cos(q2 + pi/2)*sin(q1))))/81129638414606681695789005144064 - sin(q4)*(cos(q3)*((4967757600021511*cos(q1)*sin(q2 + pi/2))/81129638414606681695789005144064 + cos(q2 + pi/2)*sin(q1)) + sin(q3)*((4967757600021511*cos(q1)*cos(q2 + pi/2))/81129638414606681695789005144064 - sin(q1)*sin(q2 + pi/2)))))/81129638414606681695789005144064) + cos(q6)*((24678615572571482867467662723121*cos(q1))/6582018229284824168619876730229402019930943462534319453394436096 + cos(q1)*cos(q4) - (4967757600021511*cos(q3)*((4967757600021511*cos(q1)*cos(q2 + pi/2))/81129638414606681695789005144064 - sin(q1)*sin(q2 + pi/2)))/81129638414606681695789005144064 + (4967757600021511*sin(q3)*((4967757600021511*cos(q1)*sin(q2 + pi/2))/81129638414606681695789005144064 + cos(q2 + pi/2)*sin(q1)))/81129638414606681695789005144064 + (4967757600021511*cos(q4)*(cos(q3)*((4967757600021511*cos(q1)*cos(q2 + pi/2))/81129638414606681695789005144064 - sin(q1)*sin(q2 + pi/2)) - sin(q3)*((4967757600021511*cos(q1)*sin(q2 + pi/2))/81129638414606681695789005144064 + cos(q2 + pi/2)*sin(q1))))/81129638414606681695789005144064 - sin(q4)*(cos(q3)*((4967757600021511*cos(q1)*sin(q2 + pi/2))/81129638414606681695789005144064 + cos(q2 + pi/2)*sin(q1)) + sin(q3)*((4967757600021511*cos(q1)*cos(q2 + pi/2))/81129638414606681695789005144064 - sin(q1)*sin(q2 + pi/2)))) + (4967757600021511*sin(q6)*((24678615572571482867467662723121*cos(q1))/6582018229284824168619876730229402019930943462534319453394436096 + cos(q1)*cos(q4) - (4967757600021511*cos(q3)*((4967757600021511*cos(q1)*cos(q2 + pi/2))/81129638414606681695789005144064 - sin(q1)*sin(q2 + pi/2)))/81129638414606681695789005144064 + (4967757600021511*sin(q3)*((4967757600021511*cos(q1)*sin(q2 + pi/2))/81129638414606681695789005144064 + cos(q2 + pi/2)*sin(q1)))/81129638414606681695789005144064 + (4967757600021511*cos(q4)*(cos(q3)*((4967757600021511*cos(q1)*cos(q2 + pi/2))/81129638414606681695789005144064 - sin(q1)*sin(q2 + pi/2)) - sin(q3)*((4967757600021511*cos(q1)*sin(q2 + pi/2))/81129638414606681695789005144064 + cos(q2 + pi/2)*sin(q1))))/81129638414606681695789005144064 - sin(q4)*(cos(q3)*((4967757600021511*cos(q1)*sin(q2 + pi/2))/81129638414606681695789005144064 + cos(q2 + pi/2)*sin(q1)) + sin(q3)*((4967757600021511*cos(q1)*cos(q2 + pi/2))/81129638414606681695789005144064 - sin(q1)*sin(q2 + pi/2)))))/40564819207303340847894502572032;
R(2,3)= (122597380068651197257713859414983140362437055831*cos(q1))/533996758980227520598755426542388028650676130589163192486760401955554931445160137505740521734144 + (4967757600021511*cos(q1)*cos(q4))/81129638414606681695789005144064 - (24678615572571482867467662723121*cos(q3)*((4967757600021511*cos(q1)*cos(q2 + pi/2))/81129638414606681695789005144064 - sin(q1)*sin(q2 + pi/2)))/6582018229284824168619876730229402019930943462534319453394436096 + (24678615572571482867467662723121*sin(q3)*((4967757600021511*cos(q1)*sin(q2 + pi/2))/81129638414606681695789005144064 + cos(q2 + pi/2)*sin(q1)))/6582018229284824168619876730229402019930943462534319453394436096 + cos(q5)*((4967757600021511*cos(q1))/81129638414606681695789005144064 - cos(q3)*((4967757600021511*cos(q1)*cos(q2 + pi/2))/81129638414606681695789005144064 - sin(q1)*sin(q2 + pi/2)) + sin(q3)*((4967757600021511*cos(q1)*sin(q2 + pi/2))/81129638414606681695789005144064 + cos(q2 + pi/2)*sin(q1))) - (4967757600021511*cos(q5)*(cos(q1)*cos(q4) + (4967757600021511*cos(q4)*(cos(q3)*((4967757600021511*cos(q1)*cos(q2 + pi/2))/81129638414606681695789005144064 - sin(q1)*sin(q2 + pi/2)) - sin(q3)*((4967757600021511*cos(q1)*sin(q2 + pi/2))/81129638414606681695789005144064 + cos(q2 + pi/2)*sin(q1))))/81129638414606681695789005144064 - sin(q4)*(cos(q3)*((4967757600021511*cos(q1)*sin(q2 + pi/2))/81129638414606681695789005144064 + cos(q2 + pi/2)*sin(q1)) + sin(q3)*((4967757600021511*cos(q1)*cos(q2 + pi/2))/81129638414606681695789005144064 - sin(q1)*sin(q2 + pi/2)))))/81129638414606681695789005144064 + sin(q5)*(cos(q1)*sin(q4) + cos(q4)*(cos(q3)*((4967757600021511*cos(q1)*sin(q2 + pi/2))/81129638414606681695789005144064 + cos(q2 + pi/2)*sin(q1)) + sin(q3)*((4967757600021511*cos(q1)*cos(q2 + pi/2))/81129638414606681695789005144064 - sin(q1)*sin(q2 + pi/2))) + (4967757600021511*sin(q4)*(cos(q3)*((4967757600021511*cos(q1)*cos(q2 + pi/2))/81129638414606681695789005144064 - sin(q1)*sin(q2 + pi/2)) - sin(q3)*((4967757600021511*cos(q1)*sin(q2 + pi/2))/81129638414606681695789005144064 + cos(q2 + pi/2)*sin(q1))))/81129638414606681695789005144064) + (24678615572571482867467662723121*cos(q4)*(cos(q3)*((4967757600021511*cos(q1)*cos(q2 + pi/2))/81129638414606681695789005144064 - sin(q1)*sin(q2 + pi/2)) - sin(q3)*((4967757600021511*cos(q1)*sin(q2 + pi/2))/81129638414606681695789005144064 + cos(q2 + pi/2)*sin(q1))))/6582018229284824168619876730229402019930943462534319453394436096 - (4967757600021511*sin(q4)*(cos(q3)*((4967757600021511*cos(q1)*sin(q2 + pi/2))/81129638414606681695789005144064 + cos(q2 + pi/2)*sin(q1)) + sin(q3)*((4967757600021511*cos(q1)*cos(q2 + pi/2))/81129638414606681695789005144064 - sin(q1)*sin(q2 + pi/2))))/81129638414606681695789005144064;
R(3,1)= (4967757600021511*sin(q6)*((4967757600021511*cos(q5)*((4967757600021511*cos(q4))/81129638414606681695789005144064 - (4967757600021511*cos(q4)*(cos(q3)*cos(q2 + pi/2) - sin(q3)*sin(q2 + pi/2)))/81129638414606681695789005144064 + sin(q4)*(cos(q3)*sin(q2 + pi/2) + cos(q2 + pi/2)*sin(q3))))/81129638414606681695789005144064 + sin(q5)*(cos(q4)*(cos(q3)*sin(q2 + pi/2) + cos(q2 + pi/2)*sin(q3)) - (4967757600021511*sin(q4))/81129638414606681695789005144064 + (4967757600021511*sin(q4)*(cos(q3)*cos(q2 + pi/2) - sin(q3)*sin(q2 + pi/2)))/81129638414606681695789005144064) - cos(q5)*(cos(q3)*cos(q2 + pi/2) - sin(q3)*sin(q2 + pi/2) + 24678615572571482867467662723121/6582018229284824168619876730229402019930943462534319453394436096)))/81129638414606681695789005144064 - cos(q6)*(cos(q5)*(cos(q4)*(cos(q3)*sin(q2 + pi/2) + cos(q2 + pi/2)*sin(q3)) - (4967757600021511*sin(q4))/81129638414606681695789005144064 + (4967757600021511*sin(q4)*(cos(q3)*cos(q2 + pi/2) - sin(q3)*sin(q2 + pi/2)))/81129638414606681695789005144064) - (4967757600021511*sin(q5)*((4967757600021511*cos(q4))/81129638414606681695789005144064 - (4967757600021511*cos(q4)*(cos(q3)*cos(q2 + pi/2) - sin(q3)*sin(q2 + pi/2)))/81129638414606681695789005144064 + sin(q4)*(cos(q3)*sin(q2 + pi/2) + cos(q2 + pi/2)*sin(q3))))/81129638414606681695789005144064 + sin(q5)*(cos(q3)*cos(q2 + pi/2) - sin(q3)*sin(q2 + pi/2) + 24678615572571482867467662723121/6582018229284824168619876730229402019930943462534319453394436096)) - (24678615572571482867467662723121*cos(q6)*((4967757600021511*cos(q5)*((4967757600021511*cos(q4))/81129638414606681695789005144064 - (4967757600021511*cos(q4)*(cos(q3)*cos(q2 + pi/2) - sin(q3)*sin(q2 + pi/2)))/81129638414606681695789005144064 + sin(q4)*(cos(q3)*sin(q2 + pi/2) + cos(q2 + pi/2)*sin(q3))))/81129638414606681695789005144064 + sin(q5)*(cos(q4)*(cos(q3)*sin(q2 + pi/2) + cos(q2 + pi/2)*sin(q3)) - (4967757600021511*sin(q4))/81129638414606681695789005144064 + (4967757600021511*sin(q4)*(cos(q3)*cos(q2 + pi/2) - sin(q3)*sin(q2 + pi/2)))/81129638414606681695789005144064) - cos(q5)*(cos(q3)*cos(q2 + pi/2) - sin(q3)*sin(q2 + pi/2) + 24678615572571482867467662723121/6582018229284824168619876730229402019930943462534319453394436096)))/3291009114642412084309938365114701009965471731267159726697218048 - (4967757600021511*sin(q6)*(cos(q5)*(cos(q4)*(cos(q3)*sin(q2 + pi/2) + cos(q2 + pi/2)*sin(q3)) - (4967757600021511*sin(q4))/81129638414606681695789005144064 + (4967757600021511*sin(q4)*(cos(q3)*cos(q2 + pi/2) - sin(q3)*sin(q2 + pi/2)))/81129638414606681695789005144064) - (4967757600021511*sin(q5)*((4967757600021511*cos(q4))/81129638414606681695789005144064 - (4967757600021511*cos(q4)*(cos(q3)*cos(q2 + pi/2) - sin(q3)*sin(q2 + pi/2)))/81129638414606681695789005144064 + sin(q4)*(cos(q3)*sin(q2 + pi/2) + cos(q2 + pi/2)*sin(q3))))/81129638414606681695789005144064 + sin(q5)*(cos(q3)*cos(q2 + pi/2) - sin(q3)*sin(q2 + pi/2) + 24678615572571482867467662723121/6582018229284824168619876730229402019930943462534319453394436096)))/40564819207303340847894502572032 - (4967757600021511*cos(q6)*((4967757600021511*cos(q4))/81129638414606681695789005144064 + (4967757600021511*cos(q3)*cos(q2 + pi/2))/81129638414606681695789005144064 - (4967757600021511*sin(q3)*sin(q2 + pi/2))/81129638414606681695789005144064 - (4967757600021511*cos(q4)*(cos(q3)*cos(q2 + pi/2) - sin(q3)*sin(q2 + pi/2)))/81129638414606681695789005144064 + sin(q4)*(cos(q3)*sin(q2 + pi/2) + cos(q2 + pi/2)*sin(q3)) + 122597380068651197257713859414983140362437055831/533996758980227520598755426542388028650676130589163192486760401955554931445160137505740521734144))/40564819207303340847894502572032 + sin(q6)*((4967757600021511*cos(q4))/81129638414606681695789005144064 + (4967757600021511*cos(q3)*cos(q2 + pi/2))/81129638414606681695789005144064 - (4967757600021511*sin(q3)*sin(q2 + pi/2))/81129638414606681695789005144064 - (4967757600021511*cos(q4)*(cos(q3)*cos(q2 + pi/2) - sin(q3)*sin(q2 + pi/2)))/81129638414606681695789005144064 + sin(q4)*(cos(q3)*sin(q2 + pi/2) + cos(q2 + pi/2)*sin(q3)) + 122597380068651197257713859414983140362437055831/533996758980227520598755426542388028650676130589163192486760401955554931445160137505740521734144); 
R(3,2)= (4967757600021511*cos(q6)*((4967757600021511*cos(q5)*((4967757600021511*cos(q4))/81129638414606681695789005144064 - (4967757600021511*cos(q4)*(cos(q3)*cos(q2 + pi/2) - sin(q3)*sin(q2 + pi/2)))/81129638414606681695789005144064 + sin(q4)*(cos(q3)*sin(q2 + pi/2) + cos(q2 + pi/2)*sin(q3))))/81129638414606681695789005144064 + sin(q5)*(cos(q4)*(cos(q3)*sin(q2 + pi/2) + cos(q2 + pi/2)*sin(q3)) - (4967757600021511*sin(q4))/81129638414606681695789005144064 + (4967757600021511*sin(q4)*(cos(q3)*cos(q2 + pi/2) - sin(q3)*sin(q2 + pi/2)))/81129638414606681695789005144064) - cos(q5)*(cos(q3)*cos(q2 + pi/2) - sin(q3)*sin(q2 + pi/2) + 24678615572571482867467662723121/6582018229284824168619876730229402019930943462534319453394436096)))/81129638414606681695789005144064 - (4967757600021511*cos(q6)*(cos(q5)*(cos(q4)*(cos(q3)*sin(q2 + pi/2) + cos(q2 + pi/2)*sin(q3)) - (4967757600021511*sin(q4))/81129638414606681695789005144064 + (4967757600021511*sin(q4)*(cos(q3)*cos(q2 + pi/2) - sin(q3)*sin(q2 + pi/2)))/81129638414606681695789005144064) - (4967757600021511*sin(q5)*((4967757600021511*cos(q4))/81129638414606681695789005144064 - (4967757600021511*cos(q4)*(cos(q3)*cos(q2 + pi/2) - sin(q3)*sin(q2 + pi/2)))/81129638414606681695789005144064 + sin(q4)*(cos(q3)*sin(q2 + pi/2) + cos(q2 + pi/2)*sin(q3))))/81129638414606681695789005144064 + sin(q5)*(cos(q3)*cos(q2 + pi/2) - sin(q3)*sin(q2 + pi/2) + 24678615572571482867467662723121/6582018229284824168619876730229402019930943462534319453394436096)))/40564819207303340847894502572032 + (24678615572571482867467662723121*sin(q6)*((4967757600021511*cos(q5)*((4967757600021511*cos(q4))/81129638414606681695789005144064 - (4967757600021511*cos(q4)*(cos(q3)*cos(q2 + pi/2) - sin(q3)*sin(q2 + pi/2)))/81129638414606681695789005144064 + sin(q4)*(cos(q3)*sin(q2 + pi/2) + cos(q2 + pi/2)*sin(q3))))/81129638414606681695789005144064 + sin(q5)*(cos(q4)*(cos(q3)*sin(q2 + pi/2) + cos(q2 + pi/2)*sin(q3)) - (4967757600021511*sin(q4))/81129638414606681695789005144064 + (4967757600021511*sin(q4)*(cos(q3)*cos(q2 + pi/2) - sin(q3)*sin(q2 + pi/2)))/81129638414606681695789005144064) - cos(q5)*(cos(q3)*cos(q2 + pi/2) - sin(q3)*sin(q2 + pi/2) + 24678615572571482867467662723121/6582018229284824168619876730229402019930943462534319453394436096)))/3291009114642412084309938365114701009965471731267159726697218048 + sin(q6)*(cos(q5)*(cos(q4)*(cos(q3)*sin(q2 + pi/2) + cos(q2 + pi/2)*sin(q3)) - (4967757600021511*sin(q4))/81129638414606681695789005144064 + (4967757600021511*sin(q4)*(cos(q3)*cos(q2 + pi/2) - sin(q3)*sin(q2 + pi/2)))/81129638414606681695789005144064) - (4967757600021511*sin(q5)*((4967757600021511*cos(q4))/81129638414606681695789005144064 - (4967757600021511*cos(q4)*(cos(q3)*cos(q2 + pi/2) - sin(q3)*sin(q2 + pi/2)))/81129638414606681695789005144064 + sin(q4)*(cos(q3)*sin(q2 + pi/2) + cos(q2 + pi/2)*sin(q3))))/81129638414606681695789005144064 + sin(q5)*(cos(q3)*cos(q2 + pi/2) - sin(q3)*sin(q2 + pi/2) + 24678615572571482867467662723121/6582018229284824168619876730229402019930943462534319453394436096)) + cos(q6)*((4967757600021511*cos(q4))/81129638414606681695789005144064 + (4967757600021511*cos(q3)*cos(q2 + pi/2))/81129638414606681695789005144064 - (4967757600021511*sin(q3)*sin(q2 + pi/2))/81129638414606681695789005144064 - (4967757600021511*cos(q4)*(cos(q3)*cos(q2 + pi/2) - sin(q3)*sin(q2 + pi/2)))/81129638414606681695789005144064 + sin(q4)*(cos(q3)*sin(q2 + pi/2) + cos(q2 + pi/2)*sin(q3)) + 122597380068651197257713859414983140362437055831/533996758980227520598755426542388028650676130589163192486760401955554931445160137505740521734144) + (4967757600021511*sin(q6)*((4967757600021511*cos(q4))/81129638414606681695789005144064 + (4967757600021511*cos(q3)*cos(q2 + pi/2))/81129638414606681695789005144064 - (4967757600021511*sin(q3)*sin(q2 + pi/2))/81129638414606681695789005144064 - (4967757600021511*cos(q4)*(cos(q3)*cos(q2 + pi/2) - sin(q3)*sin(q2 + pi/2)))/81129638414606681695789005144064 + sin(q4)*(cos(q3)*sin(q2 + pi/2) + cos(q2 + pi/2)*sin(q3)) + 122597380068651197257713859414983140362437055831/533996758980227520598755426542388028650676130589163192486760401955554931445160137505740521734144))/40564819207303340847894502572032;
R(3,3)=  (24678615572571482867467662723121*cos(q4))/6582018229284824168619876730229402019930943462534319453394436096 - (4967757600021511*cos(q5)*((4967757600021511*cos(q4))/81129638414606681695789005144064 - (4967757600021511*cos(q4)*(cos(q3)*cos(q2 + pi/2) - sin(q3)*sin(q2 + pi/2)))/81129638414606681695789005144064 + sin(q4)*(cos(q3)*sin(q2 + pi/2) + cos(q2 + pi/2)*sin(q3))))/81129638414606681695789005144064 + (24678615572571482867467662723121*cos(q3)*cos(q2 + pi/2))/6582018229284824168619876730229402019930943462534319453394436096 - sin(q5)*(cos(q4)*(cos(q3)*sin(q2 + pi/2) + cos(q2 + pi/2)*sin(q3)) - (4967757600021511*sin(q4))/81129638414606681695789005144064 + (4967757600021511*sin(q4)*(cos(q3)*cos(q2 + pi/2) - sin(q3)*sin(q2 + pi/2)))/81129638414606681695789005144064) + cos(q5)*(cos(q3)*cos(q2 + pi/2) - sin(q3)*sin(q2 + pi/2) + 24678615572571482867467662723121/6582018229284824168619876730229402019930943462534319453394436096) - (24678615572571482867467662723121*sin(q3)*sin(q2 + pi/2))/6582018229284824168619876730229402019930943462534319453394436096 - (24678615572571482867467662723121*cos(q4)*(cos(q3)*cos(q2 + pi/2) - sin(q3)*sin(q2 + pi/2)))/6582018229284824168619876730229402019930943462534319453394436096 + (4967757600021511*sin(q4)*(cos(q3)*sin(q2 + pi/2) + cos(q2 + pi/2)*sin(q3)))/81129638414606681695789005144064 + 609034066578767699168763939638324732237239140958410949107980641/43322963970637732180912721627235682866194329302747133987038743447103457934462900359999600095377180907771737671271930809827721216;

x= d4*(cos(q3)*(cos(q1)*sin(q2 + pi/2) + (4967757600021511*cos(q2 + pi/2)*sin(q1))/81129638414606681695789005144064) + sin(q3)*(cos(q1)*cos(q2 + pi/2) - (4967757600021511*sin(q1)*sin(q2 + pi/2))/81129638414606681695789005144064)) - dee*((122597380068651197257713859414983140362437055831*sin(q1))/533996758980227520598755426542388028650676130589163192486760401955554931445160137505740521734144 - (24678615572571482867467662723121*cos(q3)*(cos(q1)*sin(q2 + pi/2) + (4967757600021511*cos(q2 + pi/2)*sin(q1))/81129638414606681695789005144064))/6582018229284824168619876730229402019930943462534319453394436096 + (4967757600021511*cos(q4)*sin(q1))/81129638414606681695789005144064 - (24678615572571482867467662723121*sin(q3)*(cos(q1)*cos(q2 + pi/2) - (4967757600021511*sin(q1)*sin(q2 + pi/2))/81129638414606681695789005144064))/6582018229284824168619876730229402019930943462534319453394436096 - cos(q5)*(cos(q3)*(cos(q1)*sin(q2 + pi/2) + (4967757600021511*cos(q2 + pi/2)*sin(q1))/81129638414606681695789005144064) - (4967757600021511*sin(q1))/81129638414606681695789005144064 + sin(q3)*(cos(q1)*cos(q2 + pi/2) - (4967757600021511*sin(q1)*sin(q2 + pi/2))/81129638414606681695789005144064)) - (4967757600021511*cos(q5)*(cos(q4)*sin(q1) + (4967757600021511*cos(q4)*(cos(q3)*(cos(q1)*sin(q2 + pi/2) + (4967757600021511*cos(q2 + pi/2)*sin(q1))/81129638414606681695789005144064) + sin(q3)*(cos(q1)*cos(q2 + pi/2) - (4967757600021511*sin(q1)*sin(q2 + pi/2))/81129638414606681695789005144064)))/81129638414606681695789005144064 + sin(q4)*(cos(q3)*(cos(q1)*cos(q2 + pi/2) - (4967757600021511*sin(q1)*sin(q2 + pi/2))/81129638414606681695789005144064) - sin(q3)*(cos(q1)*sin(q2 + pi/2) + (4967757600021511*cos(q2 + pi/2)*sin(q1))/81129638414606681695789005144064))))/81129638414606681695789005144064 + sin(q5)*(sin(q1)*sin(q4) - cos(q4)*(cos(q3)*(cos(q1)*cos(q2 + pi/2) - (4967757600021511*sin(q1)*sin(q2 + pi/2))/81129638414606681695789005144064) - sin(q3)*(cos(q1)*sin(q2 + pi/2) + (4967757600021511*cos(q2 + pi/2)*sin(q1))/81129638414606681695789005144064)) + (4967757600021511*sin(q4)*(cos(q3)*(cos(q1)*sin(q2 + pi/2) + (4967757600021511*cos(q2 + pi/2)*sin(q1))/81129638414606681695789005144064) + sin(q3)*(cos(q1)*cos(q2 + pi/2) - (4967757600021511*sin(q1)*sin(q2 + pi/2))/81129638414606681695789005144064)))/81129638414606681695789005144064) + (24678615572571482867467662723121*cos(q4)*(cos(q3)*(cos(q1)*sin(q2 + pi/2) + (4967757600021511*cos(q2 + pi/2)*sin(q1))/81129638414606681695789005144064) + sin(q3)*(cos(q1)*cos(q2 + pi/2) - (4967757600021511*sin(q1)*sin(q2 + pi/2))/81129638414606681695789005144064)))/6582018229284824168619876730229402019930943462534319453394436096 + (4967757600021511*sin(q4)*(cos(q3)*(cos(q1)*cos(q2 + pi/2) - (4967757600021511*sin(q1)*sin(q2 + pi/2))/81129638414606681695789005144064) - sin(q3)*(cos(q1)*sin(q2 + pi/2) + (4967757600021511*cos(q2 + pi/2)*sin(q1))/81129638414606681695789005144064)))/81129638414606681695789005144064) - l4*(cos(q3)*(cos(q1)*cos(q2 + pi/2) - (4967757600021511*sin(q1)*sin(q2 + pi/2))/81129638414606681695789005144064) - sin(q3)*(cos(q1)*sin(q2 + pi/2) + (4967757600021511*cos(q2 + pi/2)*sin(q1))/81129638414606681695789005144064)) - (4967757600021511*d4*sin(q1))/81129638414606681695789005144064 - l3*(cos(q1)*cos(q2 + pi/2) - (4967757600021511*sin(q1)*sin(q2 + pi/2))/81129638414606681695789005144064) + l6*(sin(q5)*(cos(q3)*(cos(q1)*sin(q2 + pi/2) + (4967757600021511*cos(q2 + pi/2)*sin(q1))/81129638414606681695789005144064) - (4967757600021511*sin(q1))/81129638414606681695789005144064 + sin(q3)*(cos(q1)*cos(q2 + pi/2) - (4967757600021511*sin(q1)*sin(q2 + pi/2))/81129638414606681695789005144064)) + (4967757600021511*sin(q5)*(cos(q4)*sin(q1) + (4967757600021511*cos(q4)*(cos(q3)*(cos(q1)*sin(q2 + pi/2) + (4967757600021511*cos(q2 + pi/2)*sin(q1))/81129638414606681695789005144064) + sin(q3)*(cos(q1)*cos(q2 + pi/2) - (4967757600021511*sin(q1)*sin(q2 + pi/2))/81129638414606681695789005144064)))/81129638414606681695789005144064 + sin(q4)*(cos(q3)*(cos(q1)*cos(q2 + pi/2) - (4967757600021511*sin(q1)*sin(q2 + pi/2))/81129638414606681695789005144064) - sin(q3)*(cos(q1)*sin(q2 + pi/2) + (4967757600021511*cos(q2 + pi/2)*sin(q1))/81129638414606681695789005144064))))/81129638414606681695789005144064 + cos(q5)*(sin(q1)*sin(q4) - cos(q4)*(cos(q3)*(cos(q1)*cos(q2 + pi/2) - (4967757600021511*sin(q1)*sin(q2 + pi/2))/81129638414606681695789005144064) - sin(q3)*(cos(q1)*sin(q2 + pi/2) + (4967757600021511*cos(q2 + pi/2)*sin(q1))/81129638414606681695789005144064)) + (4967757600021511*sin(q4)*(cos(q3)*(cos(q1)*sin(q2 + pi/2) + (4967757600021511*cos(q2 + pi/2)*sin(q1))/81129638414606681695789005144064) + sin(q3)*(cos(q1)*cos(q2 + pi/2) - (4967757600021511*sin(q1)*sin(q2 + pi/2))/81129638414606681695789005144064)))/81129638414606681695789005144064));
y= (4967757600021511*d4*cos(q1))/81129638414606681695789005144064 - l4*(cos(q3)*((4967757600021511*cos(q1)*sin(q2 + pi/2))/81129638414606681695789005144064 + cos(q2 + pi/2)*sin(q1)) + sin(q3)*((4967757600021511*cos(q1)*cos(q2 + pi/2))/81129638414606681695789005144064 - sin(q1)*sin(q2 + pi/2))) - d4*(cos(q3)*((4967757600021511*cos(q1)*cos(q2 + pi/2))/81129638414606681695789005144064 - sin(q1)*sin(q2 + pi/2)) - sin(q3)*((4967757600021511*cos(q1)*sin(q2 + pi/2))/81129638414606681695789005144064 + cos(q2 + pi/2)*sin(q1))) - l3*((4967757600021511*cos(q1)*sin(q2 + pi/2))/81129638414606681695789005144064 + cos(q2 + pi/2)*sin(q1)) - l6*(cos(q5)*(cos(q1)*sin(q4) + cos(q4)*(cos(q3)*((4967757600021511*cos(q1)*sin(q2 + pi/2))/81129638414606681695789005144064 + cos(q2 + pi/2)*sin(q1)) + sin(q3)*((4967757600021511*cos(q1)*cos(q2 + pi/2))/81129638414606681695789005144064 - sin(q1)*sin(q2 + pi/2))) + (4967757600021511*sin(q4)*(cos(q3)*((4967757600021511*cos(q1)*cos(q2 + pi/2))/81129638414606681695789005144064 - sin(q1)*sin(q2 + pi/2)) - sin(q3)*((4967757600021511*cos(q1)*sin(q2 + pi/2))/81129638414606681695789005144064 + cos(q2 + pi/2)*sin(q1))))/81129638414606681695789005144064) - sin(q5)*((4967757600021511*cos(q1))/81129638414606681695789005144064 - cos(q3)*((4967757600021511*cos(q1)*cos(q2 + pi/2))/81129638414606681695789005144064 - sin(q1)*sin(q2 + pi/2)) + sin(q3)*((4967757600021511*cos(q1)*sin(q2 + pi/2))/81129638414606681695789005144064 + cos(q2 + pi/2)*sin(q1))) + (4967757600021511*sin(q5)*(cos(q1)*cos(q4) + (4967757600021511*cos(q4)*(cos(q3)*((4967757600021511*cos(q1)*cos(q2 + pi/2))/81129638414606681695789005144064 - sin(q1)*sin(q2 + pi/2)) - sin(q3)*((4967757600021511*cos(q1)*sin(q2 + pi/2))/81129638414606681695789005144064 + cos(q2 + pi/2)*sin(q1))))/81129638414606681695789005144064 - sin(q4)*(cos(q3)*((4967757600021511*cos(q1)*sin(q2 + pi/2))/81129638414606681695789005144064 + cos(q2 + pi/2)*sin(q1)) + sin(q3)*((4967757600021511*cos(q1)*cos(q2 + pi/2))/81129638414606681695789005144064 - sin(q1)*sin(q2 + pi/2)))))/81129638414606681695789005144064) + dee*((122597380068651197257713859414983140362437055831*cos(q1))/533996758980227520598755426542388028650676130589163192486760401955554931445160137505740521734144 + (4967757600021511*cos(q1)*cos(q4))/81129638414606681695789005144064 - (24678615572571482867467662723121*cos(q3)*((4967757600021511*cos(q1)*cos(q2 + pi/2))/81129638414606681695789005144064 - sin(q1)*sin(q2 + pi/2)))/6582018229284824168619876730229402019930943462534319453394436096 + (24678615572571482867467662723121*sin(q3)*((4967757600021511*cos(q1)*sin(q2 + pi/2))/81129638414606681695789005144064 + cos(q2 + pi/2)*sin(q1)))/6582018229284824168619876730229402019930943462534319453394436096 + cos(q5)*((4967757600021511*cos(q1))/81129638414606681695789005144064 - cos(q3)*((4967757600021511*cos(q1)*cos(q2 + pi/2))/81129638414606681695789005144064 - sin(q1)*sin(q2 + pi/2)) + sin(q3)*((4967757600021511*cos(q1)*sin(q2 + pi/2))/81129638414606681695789005144064 + cos(q2 + pi/2)*sin(q1))) - (4967757600021511*cos(q5)*(cos(q1)*cos(q4) + (4967757600021511*cos(q4)*(cos(q3)*((4967757600021511*cos(q1)*cos(q2 + pi/2))/81129638414606681695789005144064 - sin(q1)*sin(q2 + pi/2)) - sin(q3)*((4967757600021511*cos(q1)*sin(q2 + pi/2))/81129638414606681695789005144064 + cos(q2 + pi/2)*sin(q1))))/81129638414606681695789005144064 - sin(q4)*(cos(q3)*((4967757600021511*cos(q1)*sin(q2 + pi/2))/81129638414606681695789005144064 + cos(q2 + pi/2)*sin(q1)) + sin(q3)*((4967757600021511*cos(q1)*cos(q2 + pi/2))/81129638414606681695789005144064 - sin(q1)*sin(q2 + pi/2)))))/81129638414606681695789005144064 + sin(q5)*(cos(q1)*sin(q4) + cos(q4)*(cos(q3)*((4967757600021511*cos(q1)*sin(q2 + pi/2))/81129638414606681695789005144064 + cos(q2 + pi/2)*sin(q1)) + sin(q3)*((4967757600021511*cos(q1)*cos(q2 + pi/2))/81129638414606681695789005144064 - sin(q1)*sin(q2 + pi/2))) + (4967757600021511*sin(q4)*(cos(q3)*((4967757600021511*cos(q1)*cos(q2 + pi/2))/81129638414606681695789005144064 - sin(q1)*sin(q2 + pi/2)) - sin(q3)*((4967757600021511*cos(q1)*sin(q2 + pi/2))/81129638414606681695789005144064 + cos(q2 + pi/2)*sin(q1))))/81129638414606681695789005144064) + (24678615572571482867467662723121*cos(q4)*(cos(q3)*((4967757600021511*cos(q1)*cos(q2 + pi/2))/81129638414606681695789005144064 - sin(q1)*sin(q2 + pi/2)) - sin(q3)*((4967757600021511*cos(q1)*sin(q2 + pi/2))/81129638414606681695789005144064 + cos(q2 + pi/2)*sin(q1))))/6582018229284824168619876730229402019930943462534319453394436096 - (4967757600021511*sin(q4)*(cos(q3)*((4967757600021511*cos(q1)*sin(q2 + pi/2))/81129638414606681695789005144064 + cos(q2 + pi/2)*sin(q1)) + sin(q3)*((4967757600021511*cos(q1)*cos(q2 + pi/2))/81129638414606681695789005144064 - sin(q1)*sin(q2 + pi/2))))/81129638414606681695789005144064);
z= d1 + (24678615572571482867467662723121*d4)/6582018229284824168619876730229402019930943462534319453394436096 + dee*((24678615572571482867467662723121*cos(q4))/6582018229284824168619876730229402019930943462534319453394436096 - (4967757600021511*cos(q5)*((4967757600021511*cos(q4))/81129638414606681695789005144064 - (4967757600021511*cos(q4)*(cos(q3)*cos(q2 + pi/2) - sin(q3)*sin(q2 + pi/2)))/81129638414606681695789005144064 + sin(q4)*(cos(q3)*sin(q2 + pi/2) + cos(q2 + pi/2)*sin(q3))))/81129638414606681695789005144064 + (24678615572571482867467662723121*cos(q3)*cos(q2 + pi/2))/6582018229284824168619876730229402019930943462534319453394436096 - sin(q5)*(cos(q4)*(cos(q3)*sin(q2 + pi/2) + cos(q2 + pi/2)*sin(q3)) - (4967757600021511*sin(q4))/81129638414606681695789005144064 + (4967757600021511*sin(q4)*(cos(q3)*cos(q2 + pi/2) - sin(q3)*sin(q2 + pi/2)))/81129638414606681695789005144064) + cos(q5)*(cos(q3)*cos(q2 + pi/2) - sin(q3)*sin(q2 + pi/2) + 24678615572571482867467662723121/6582018229284824168619876730229402019930943462534319453394436096) - (24678615572571482867467662723121*sin(q3)*sin(q2 + pi/2))/6582018229284824168619876730229402019930943462534319453394436096 - (24678615572571482867467662723121*cos(q4)*(cos(q3)*cos(q2 + pi/2) - sin(q3)*sin(q2 + pi/2)))/6582018229284824168619876730229402019930943462534319453394436096 + (4967757600021511*sin(q4)*(cos(q3)*sin(q2 + pi/2) + cos(q2 + pi/2)*sin(q3)))/81129638414606681695789005144064 + 609034066578767699168763939638324732237239140958410949107980641/43322963970637732180912721627235682866194329302747133987038743447103457934462900359999600095377180907771737671271930809827721216) + d4*(cos(q3)*cos(q2 + pi/2) - sin(q3)*sin(q2 + pi/2)) + l4*(cos(q3)*sin(q2 + pi/2) + cos(q2 + pi/2)*sin(q3)) + l3*sin(q2 + pi/2) + l6*(cos(q5)*(cos(q4)*(cos(q3)*sin(q2 + pi/2) + cos(q2 + pi/2)*sin(q3)) - (4967757600021511*sin(q4))/81129638414606681695789005144064 + (4967757600021511*sin(q4)*(cos(q3)*cos(q2 + pi/2) - sin(q3)*sin(q2 + pi/2)))/81129638414606681695789005144064) - (4967757600021511*sin(q5)*((4967757600021511*cos(q4))/81129638414606681695789005144064 - (4967757600021511*cos(q4)*(cos(q3)*cos(q2 + pi/2) - sin(q3)*sin(q2 + pi/2)))/81129638414606681695789005144064 + sin(q4)*(cos(q3)*sin(q2 + pi/2) + cos(q2 + pi/2)*sin(q3))))/81129638414606681695789005144064 + sin(q5)*(cos(q3)*cos(q2 + pi/2) - sin(q3)*sin(q2 + pi/2) + 24678615572571482867467662723121/6582018229284824168619876730229402019930943462534319453394436096));
end
